simulink model "kalman_beginner_temperature"  (R2025b)
settings: Solver=FixedStepDiscrete  StartTime=0.0  StopTime=30  FixedStep=0.1  RelTol=1e-3
settings Model: Creator=alosw  LastModifiedBy=alosw

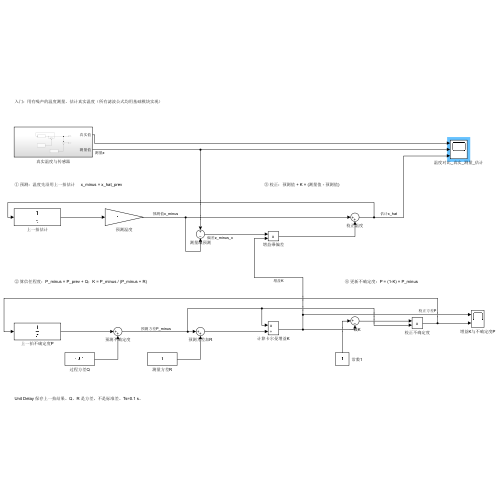
[thumbnail: Simulink's stored preview of the top-level diagram]
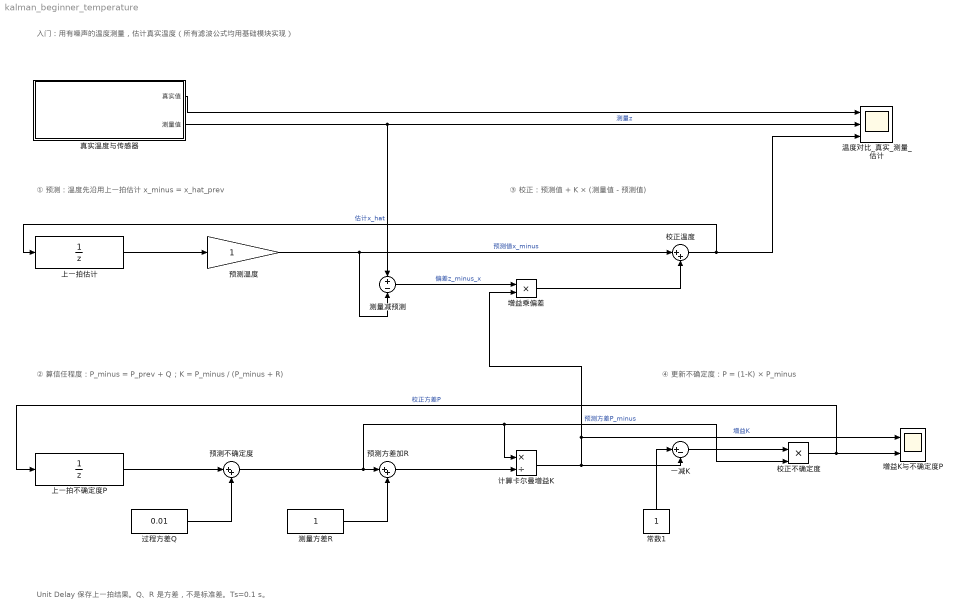
== system kalman_beginner_temperature ==
  note: 入门：用有噪声的温度测量，估计真实温度（所有滤波公式均用基础模块实现）
  note: ① 预测：温度先沿用上一拍估计 x_minus = x_hat_prev
  note: ③ 校正：预测值 + K × (测量值 - 预测值)
  note: ② 算信任程度：P_minus = P_prev + Q；K = P_minus / (P_minus + R)
  note: ④ 更新不确定度：P = (1-K) × P_minus
  note: Unit Delay 保存上一拍结果。Q、R 是方差，不是标准差。Ts=0.1 s。
  一减K : Sum  Inputs=|+-
  上一拍不确定度P : UnitDelay  InitialCondition=4  SampleTime=0.1  HasFrameUpgradeWarning=on
  上一拍估计 : UnitDelay  InitialCondition=18  SampleTime=0.1  HasFrameUpgradeWarning=on
  增益K与不确定度P : Scope  NumInputPorts=2
  增益乘偏差 : Product  Inputs=**
  常数1 : Constant
  校正不确定度 : Product  Inputs=**
  校正温度 : Sum  Inputs=|++
  测量减预测 : Sum  Inputs=+-
  测量方差R : Constant
  温度对比_真实_测量_估计 : Scope  NumInputPorts=3
      settings: ActiveDisplayYMinimum=16.417596674266072  ActiveDisplayYMaximum=25.427672860904242
  真实温度与传感器 : Subsystem
  计算卡尔曼增益K : Product  Inputs=*/
  过程方差Q : Constant  Value=0.01
  预测不确定度 : Sum  Inputs=|++
  预测方差加R : Sum  Inputs=|++
  预测温度 : Gain
  wires:
  真实温度与传感器/1(真实值) -> 温度对比_真实_测量_估计/1
  真实温度与传感器/2(测量值) -> 温度对比_真实_测量_估计/2, 测量减预测/1  "测量z"
  上一拍估计/1 -> 预测温度/1
  预测温度/1 -> 校正温度/1, 测量减预测/2  "预测值x_minus"
  测量减预测/1 -> 增益乘偏差/1  "偏差z_minus_x"
  计算卡尔曼增益K/1 -> 一减K/2, 增益K与不确定度P/1, 增益乘偏差/2  "增益K"
  增益乘偏差/1 -> 校正温度/2
  校正温度/1 -> 上一拍估计/1, 温度对比_真实_测量_估计/3  "估计x_hat"
  上一拍不确定度P/1 -> 预测不确定度/1
  过程方差Q/1 -> 预测不确定度/2
  预测不确定度/1 -> 计算卡尔曼增益K/1, 校正不确定度/2, 预测方差加R/1  "预测方差P_minus"
  测量方差R/1 -> 预测方差加R/2
  预测方差加R/1 -> 计算卡尔曼增益K/2
  常数1/1 -> 一减K/1
  一减K/1 -> 校正不确定度/1
  校正不确定度/1 -> 上一拍不确定度P/1, 增益K与不确定度P/2  "校正方差P"

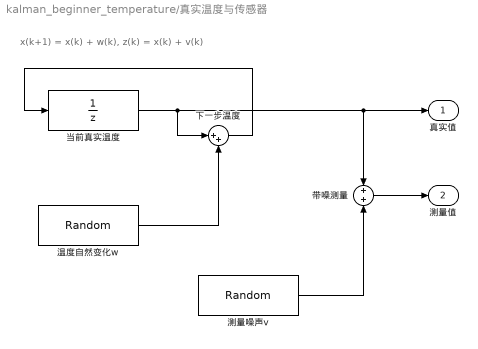
== system kalman_beginner_temperature/真实温度与传感器 ==
  note: x(k+1) = x(k) + w(k), z(k) = x(k) + v(k)
  下一步温度 : Sum  Inputs=|++
  带噪测量 : Sum
  当前真实温度 : UnitDelay  InitialCondition=20  SampleTime=0.1  HasFrameUpgradeWarning=on
  测量噪声v : RandomNumber  Seed=5678  SampleTime=0.1
  温度自然变化w : RandomNumber  Variance=0.01  Seed=1234  SampleTime=0.1
  真实值 : Outport
  测量值 : Outport  Port=2
  wires:
  当前真实温度/1 -> 真实值/1, 带噪测量/1, 下一步温度/1
  温度自然变化w/1 -> 下一步温度/2
  下一步温度/1 -> 当前真实温度/1
  测量噪声v/1 -> 带噪测量/2
  带噪测量/1 -> 测量值/1
